simulink library "fmCopterAttiRedIndi_lib"  (R2018b)
settings: Solver=VariableStepAuto  StartTime=0.0  StopTime=10.0  RelTol=1e-3
undefined symbols (not defined in the file or in its folder): fm_atti
libraries: filters_lib x2, simulink x1, ca_lib x1, cntrlAttiRedIndi_lib x1
settings Model: Creator=Ybeyer  LastModifiedBy=yannic
settings SFSimCC: SimUseLocalCustomCode=off
settings RTWCC: RTWUseLocalCustomCode=off
settings CodeAppCC: StateflowObjectComments=on

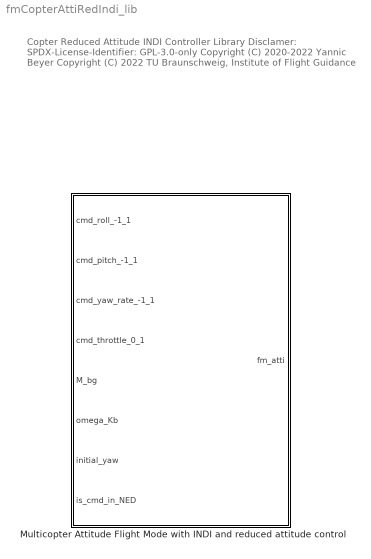
== system fmCopterAttiRedIndi_lib ==
  note: Copter Reduced Attitude INDI Controller Library
      |
      | Disclamer:
      | SPDX-License-Identifier: GPL-3.0-only
      |
      | Copyright (C) 2020-2022 Yannic Beyer
      | Copyright (C) 2022 TU Braunschweig, Institute of Flight Guidance
  Multicopter Attitude Flight Mode with INDI and reduced attitude control : Subsystem  mask{fm=fm_atti}
      mask prompts: fm "Copter Attitude Flight Mode (INDI) parameters struct, see fmCopterAttiIndi_params_default"
      mask DialogControl DescGroupVar Prompt: Multicopter Attitude Flight Mode with INDI and reduced attitude control
      mask DialogControl DescTextVar Prompt: Controller is basically implemented according to [1]
      mask DialogControl Control2 Prompt: [1] Sun, S., Baert, M., Van Schijndel, B. S., & De Visser, C. (2020, May). Upset Recovery Control for Quadrotors Subjected to a Complete Rotor Failure from Large Initial Disturbances. In 2020 IEEE International Conference on Robotics and Automation (ICRA) (pp. 4273-4279). IEEE.

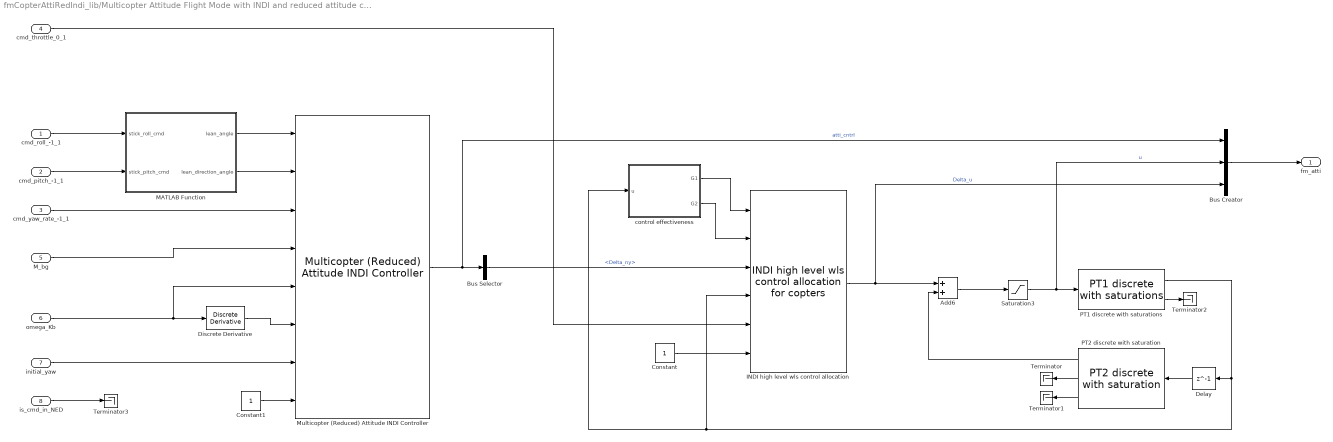
== system fmCopterAttiRedIndi_lib/Multicopter Attitude Flight Mode with INDI and reduced attitude control ==
  cmd_roll_-1_1 : Inport  SampleTime=fm.sample_time
  cmd_pitch_-1_1 : Inport  Port=2  SampleTime=fm.sample_time
  cmd_yaw_rate_-1_1 : Inport  Port=3  SampleTime=fm.sample_time
  cmd_throttle_0_1 : Inport  Port=4  SampleTime=fm.sample_time
  M_bg : Inport  Port=5  SampleTime=fm.sample_time
  omega_Kb : Inport  Port=6  SampleTime=fm.sample_time
  initial_yaw : Inport  Port=7  SampleTime=fm.sample_time
  is_cmd_in_NED : Inport  Port=8  SampleTime=fm.sample_time
  Add6 : Sum
  Bus Creator : BusCreator  Inputs=3
  Bus Selector : BusSelector  OutputSignals=pseudo_control.Delta_ny
  Constant : Constant  OutDataTypeStr=Inherit: Inherit via back propagation
  Constant1 : Constant  OutDataTypeStr=Inherit: Inherit via back propagation
  Delay : Delay  DelayLength=1
  Discrete Derivative : simulink/Discrete/Discrete Derivative  gainval=1.0  ICPrevScaledInput=0.0  OutMin=[]  OutMax=[]  OutDataType=fixdt(1, 16)  OutScaling=2^-10  DoSatur=off
  INDI high level wls control allocation : ca_lib/INDI high level wls control allocation for copters  ca=fm.ca  is_Delta_W_v_check=off  is_W_check=off  is_iter_check=off
  MATLAB Function : MATLAB Function  TreatAsAtomicUnit=on
  Multicopter (Reduced) Attitude INDI Controller : cntrlAttiRedIndi_lib/Multicopter (Reduced) Attitude INDI Controller  atc=fm.atc  T=2/fm.sens_filt.omega + fm.motor_time_constant
  PT1 discrete with saturations : filters_lib/PT1 discrete with saturations  T=fm.motor_time_constant  x_max=inf  x_min=-inf  x_dt_max=inf  x_dt_min=-inf  x_init=0
      settings: SourceProductName=LADAC
  PT2 discrete with saturation : filters_lib/PT2 discrete with saturation  omega=fm.sens_filt.omega  d=fm.sens_filt.D  x_dt2_max=inf  x_dt2_min=-inf  x_dt_max=inf  x_dt_min=-inf  x_max=inf  x_min=-inf  x_init=0  x_dt_init=0
      settings: SourceProductName=LADAC
  Saturation3 : Saturate  UpperLimit=fm.ca.u_max  LowerLimit=fm.ca.u_min
  Terminator{,1..3} (4 alike) : Terminator
  control effectiveness : Subsystem
  fm_atti : Outport  SampleTime=fm.sample_time
  wires:
  Delay/1 -> PT2 discrete with saturation/1
  PT1 discrete with saturations/1 -> INDI high level wls control allocation/4, control effectiveness/1(u), Delay/1
  initial_yaw/1 -> Multicopter (Reduced) Attitude INDI Controller/7
  cmd_pitch_-1_1/1 -> MATLAB Function/2(stick_pitch_cmd)
  cmd_yaw_rate_-1_1/1 -> Multicopter (Reduced) Attitude INDI Controller/3
  cmd_throttle_0_1/1 -> INDI high level wls control allocation/5
  Constant/1 -> INDI high level wls control allocation/6
  cmd_roll_-1_1/1 -> MATLAB Function/1(stick_roll_cmd)
  control effectiveness/2(G2) -> INDI high level wls control allocation/2
  Add6/1 -> Saturation3/1
  Multicopter (Reduced) Attitude INDI Controller/1 -> Bus Creator/1, Bus Selector/1  "atti_cntrl"
  Bus Selector/1 -> INDI high level wls control allocation/3  "<Delta_ny>"
  control effectiveness/1(G1) -> INDI high level wls control allocation/1
  Saturation3/1 -> Bus Creator/2, PT1 discrete with saturations/1  "u"
  INDI high level wls control allocation/1 -> Bus Creator/3, Add6/1  "Delta_u"
  M_bg/1 -> Multicopter (Reduced) Attitude INDI Controller/4
  omega_Kb/1 -> Discrete Derivative/1, Multicopter (Reduced) Attitude INDI Controller/5
  Discrete Derivative/1 -> Multicopter (Reduced) Attitude INDI Controller/6
  PT2 discrete with saturation/2 -> Terminator/1
  PT2 discrete with saturation/3 -> Terminator1/1
  PT1 discrete with saturations/2 -> Terminator2/1
  Bus Creator/1 -> fm_atti/1
  MATLAB Function/1(lean_angle) -> Multicopter (Reduced) Attitude INDI Controller/1
  MATLAB Function/2(lean_direction_angle) -> Multicopter (Reduced) Attitude INDI Controller/2
  Constant1/1 -> Multicopter (Reduced) Attitude INDI Controller/8
  is_cmd_in_NED/1 -> Terminator3/1
  PT2 discrete with saturation/1 -> Add6/2

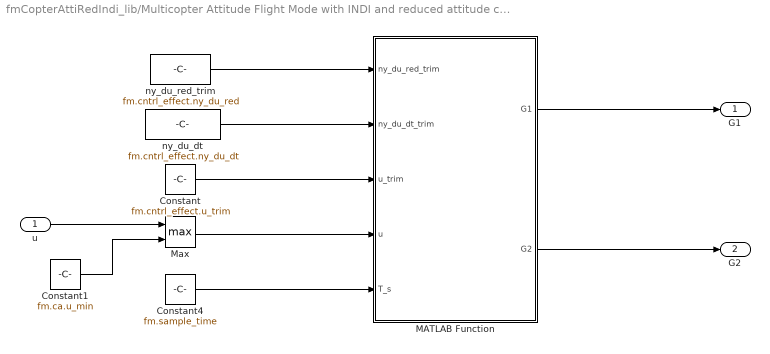
== system fmCopterAttiRedIndi_lib/Multicopter Attitude Flight Mode with INDI and reduced attitude control/control effectiveness ==
  u : Inport
  Constant : Constant  Value=fm.cntrl_effect.u_trim
  Constant1 : Constant  Value=fm.ca.u_min
  Constant4 : Constant  Value=fm.sample_time
  MATLAB Function : MATLAB Function  TreatAsAtomicUnit=on
  Max : MinMax  Function=max  Inputs=2
  ny_du_dt : Constant  Value=fm.cntrl_effect.ny_du_dt
  ny_du_red_trim : Constant  Value=fm.cntrl_effect.ny_du_red
  G1 : Outport
  G2 : Outport  Port=2
  wires:
  MATLAB Function/2(G2) -> G2/1
  MATLAB Function/1(G1) -> G1/1
  Max/1 -> MATLAB Function/4(u)
  Constant1/1 -> Max/2
  u/1 -> Max/1
  ny_du_dt/1 -> MATLAB Function/2(ny_du_dt_trim)
  Constant/1 -> MATLAB Function/3(u_trim)
  Constant4/1 -> MATLAB Function/5(T_s)
  ny_du_red_trim/1 -> MATLAB Function/1(ny_du_red_trim)

== matlab function fmCopterAttiRedIndi_lib/Multicopter Attitude Flight Mode with INDI and reduced attitude control/control effectiveness/MATLAB Function ==
  data: ny_du_red_trim input; ny_du_dt_trim input; u_trim input; u input; G1 output; T_s input; G2 output
function [G1,G2] = controlEffectiveness2G1G2( ny_du_red_trim, ny_du_dt_trim, u_trim, u, T_s) %#codegen
[G1,G2] = controlEffectiveness2G1G2( ny_du_red_trim, ny_du_dt_trim, u_trim, u, T_s);
end

== matlab function fmCopterAttiRedIndi_lib/Multicopter Attitude Flight Mode with INDI and reduced attitude control/MATLAB Function ==
  data: stick_roll_cmd input; lean_angle output; stick_pitch_cmd input; lean_direction_angle output
function [lean_angle,lean_direction_angle] = fcn(stick_roll_cmd,stick_pitch_cmd)

lean_angle = sqrt( stick_roll_cmd^2 + stick_pitch_cmd^2 );
lean_direction_angle = atan2(stick_roll_cmd,-stick_pitch_cmd);

end
